simulink model "AXU5EV_PL_Algorithm_Library"  (R2026b)
settings: Solver=VariableStepAuto
settings Model: Creator=lww  LastModifiedBy=lww

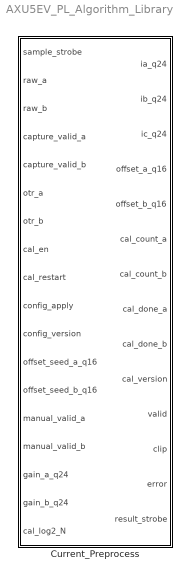
== system AXU5EV_PL_Algorithm_Library ==
  Current_Preprocess : Subsystem

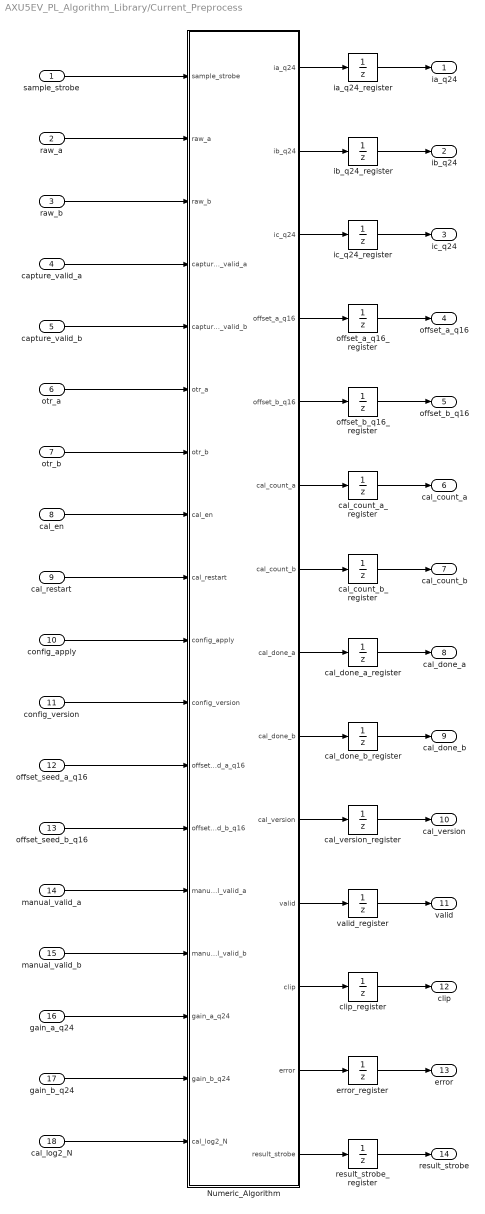
== system AXU5EV_PL_Algorithm_Library/Current_Preprocess ==
  sample_strobe : Inport  OutDataTypeStr=boolean  SampleTime=2e-8
  raw_a : Inport  Port=2  OutDataTypeStr=uint16  SampleTime=2e-8
  raw_b : Inport  Port=3  OutDataTypeStr=uint16  SampleTime=2e-8
  capture_valid_a : Inport  Port=4  OutDataTypeStr=boolean  SampleTime=2e-8
  capture_valid_b : Inport  Port=5  OutDataTypeStr=boolean  SampleTime=2e-8
  otr_a : Inport  Port=6  OutDataTypeStr=boolean  SampleTime=2e-8
  otr_b : Inport  Port=7  OutDataTypeStr=boolean  SampleTime=2e-8
  cal_en : Inport  Port=8  OutDataTypeStr=boolean  SampleTime=2e-8
  cal_restart : Inport  Port=9  OutDataTypeStr=boolean  SampleTime=2e-8
  config_apply : Inport  Port=10  OutDataTypeStr=boolean  SampleTime=2e-8
  config_version : Inport  Port=11  OutDataTypeStr=uint32  SampleTime=2e-8
  offset_seed_a_q16 : Inport  Port=12  OutDataTypeStr=int32  SampleTime=2e-8
  offset_seed_b_q16 : Inport  Port=13  OutDataTypeStr=int32  SampleTime=2e-8
  manual_valid_a : Inport  Port=14  OutDataTypeStr=boolean  SampleTime=2e-8
  manual_valid_b : Inport  Port=15  OutDataTypeStr=boolean  SampleTime=2e-8
  gain_a_q24 : Inport  Port=16  OutDataTypeStr=int32  SampleTime=2e-8
  gain_b_q24 : Inport  Port=17  OutDataTypeStr=int32  SampleTime=2e-8
  cal_log2_N : Inport  Port=18  OutDataTypeStr=uint8  SampleTime=2e-8
  Numeric_Algorithm : MATLAB Function  TreatAsAtomicUnit=on
  cal_count_a_register : UnitDelay  SampleTime=-1
  cal_count_b_register : UnitDelay  SampleTime=-1
  cal_done_a_register : UnitDelay  SampleTime=-1
  cal_done_b_register : UnitDelay  SampleTime=-1
  cal_version_register : UnitDelay  SampleTime=-1
  clip_register : UnitDelay  SampleTime=-1
  error_register : UnitDelay  SampleTime=-1
  ia_q24_register : UnitDelay  SampleTime=-1
  ib_q24_register : UnitDelay  SampleTime=-1
  ic_q24_register : UnitDelay  SampleTime=-1
  offset_a_q16_register : UnitDelay  SampleTime=-1
  offset_b_q16_register : UnitDelay  SampleTime=-1
  result_strobe_register : UnitDelay  SampleTime=-1
  valid_register : UnitDelay  SampleTime=-1
  ia_q24 : Outport  OutDataTypeStr=int32
  ib_q24 : Outport  Port=2  OutDataTypeStr=int32
  ic_q24 : Outport  Port=3  OutDataTypeStr=int32
  offset_a_q16 : Outport  Port=4  OutDataTypeStr=int32
  offset_b_q16 : Outport  Port=5  OutDataTypeStr=int32
  cal_count_a : Outport  Port=6  OutDataTypeStr=uint16
  cal_count_b : Outport  Port=7  OutDataTypeStr=uint16
  cal_done_a : Outport  Port=8  OutDataTypeStr=boolean
  cal_done_b : Outport  Port=9  OutDataTypeStr=boolean
  cal_version : Outport  Port=10  OutDataTypeStr=uint32
  valid : Outport  Port=11  OutDataTypeStr=boolean
  clip : Outport  Port=12  OutDataTypeStr=boolean
  error : Outport  Port=13  OutDataTypeStr=uint16
  result_strobe : Outport  Port=14  OutDataTypeStr=boolean
  wires:
  result_strobe_register/1 -> result_strobe/1
  error_register/1 -> error/1
  clip_register/1 -> clip/1
  valid_register/1 -> valid/1
  cal_version_register/1 -> cal_version/1
  cal_done_b_register/1 -> cal_done_b/1
  cal_done_a_register/1 -> cal_done_a/1
  cal_count_b_register/1 -> cal_count_b/1
  cal_count_a_register/1 -> cal_count_a/1
  offset_b_q16_register/1 -> offset_b_q16/1
  offset_a_q16_register/1 -> offset_a_q16/1
  ic_q24_register/1 -> ic_q24/1
  ib_q24_register/1 -> ib_q24/1
  ia_q24_register/1 -> ia_q24/1
  Numeric_Algorithm/1(ia_q24) -> ia_q24_register/1
  sample_strobe/1 -> Numeric_Algorithm/1(sample_strobe)
  raw_a/1 -> Numeric_Algorithm/2(raw_a)
  raw_b/1 -> Numeric_Algorithm/3(raw_b)
  capture_valid_a/1 -> Numeric_Algorithm/4(capture_valid_a)
  capture_valid_b/1 -> Numeric_Algorithm/5(capture_valid_b)
  otr_a/1 -> Numeric_Algorithm/6(otr_a)
  otr_b/1 -> Numeric_Algorithm/7(otr_b)
  cal_en/1 -> Numeric_Algorithm/8(cal_en)
  cal_restart/1 -> Numeric_Algorithm/9(cal_restart)
  config_apply/1 -> Numeric_Algorithm/10(config_apply)
  config_version/1 -> Numeric_Algorithm/11(config_version)
  offset_seed_a_q16/1 -> Numeric_Algorithm/12(offset_seed_a_q16)
  offset_seed_b_q16/1 -> Numeric_Algorithm/13(offset_seed_b_q16)
  manual_valid_a/1 -> Numeric_Algorithm/14(manual_valid_a)
  manual_valid_b/1 -> Numeric_Algorithm/15(manual_valid_b)
  gain_a_q24/1 -> Numeric_Algorithm/16(gain_a_q24)
  gain_b_q24/1 -> Numeric_Algorithm/17(gain_b_q24)
  cal_log2_N/1 -> Numeric_Algorithm/18(cal_log2_N)
  Numeric_Algorithm/2(ib_q24) -> ib_q24_register/1
  Numeric_Algorithm/3(ic_q24) -> ic_q24_register/1
  Numeric_Algorithm/4(offset_a_q16) -> offset_a_q16_register/1
  Numeric_Algorithm/5(offset_b_q16) -> offset_b_q16_register/1
  Numeric_Algorithm/6(cal_count_a) -> cal_count_a_register/1
  Numeric_Algorithm/7(cal_count_b) -> cal_count_b_register/1
  Numeric_Algorithm/8(cal_done_a) -> cal_done_a_register/1
  Numeric_Algorithm/9(cal_done_b) -> cal_done_b_register/1
  Numeric_Algorithm/10(cal_version) -> cal_version_register/1
  Numeric_Algorithm/11(valid) -> valid_register/1
  Numeric_Algorithm/12(clip) -> clip_register/1
  Numeric_Algorithm/13(error) -> error_register/1
  Numeric_Algorithm/14(result_strobe) -> result_strobe_register/1

== matlab function AXU5EV_PL_Algorithm_Library/Current_Preprocess/Numeric_Algorithm ==
  data: sample_strobe input; ia_q24 output; raw_a input; raw_b input; capture_valid_a input; capture_valid_b input; otr_a input; otr_b input; cal_en input; cal_restart input; config_apply input; config_version input; offset_seed_a_q16 input; offset_seed_b_q16 input; manual_valid_a input; manual_valid_b input; gain_a_q24 input; gain_b_q24 input; cal_log2_N input; ib_q24 output; ic_q24 output; offset_a_q16 output; offset_b_q16 output; cal_count_a output; cal_count_b output; cal_done_a output; cal_done_b output; cal_version output; valid output; clip output; error output; result_strobe output
function [ia_q24,ib_q24,ic_q24,offset_a_q16,offset_b_q16,cal_count_a,cal_count_b,cal_done_a,cal_done_b,cal_version,valid,clip,error,result_strobe] = f(sample_strobe,raw_a,raw_b,capture_valid_a,capture_valid_b,otr_a,otr_b,cal_en,cal_restart,config_apply,config_version,offset_seed_a_q16,offset_seed_b_q16,manual_valid_a,manual_valid_b,gain_a_q24,gain_b_q24,cal_log2_N)
%#codegen
[ia_q24,ib_q24,ic_q24,offset_a_q16,offset_b_q16,cal_count_a,cal_count_b,cal_done_a,cal_done_b,cal_version,valid,clip,error,result_strobe] = ax03b1_current_preprocess(sample_strobe,raw_a,raw_b,capture_valid_a,capture_valid_b,otr_a,otr_b,cal_en,cal_restart,config_apply,config_version,offset_seed_a_q16,offset_seed_b_q16,manual_valid_a,manual_valid_b,gain_a_q24,gain_b_q24,cal_log2_N);
end
